simulink model "RIPS_model_pil"  (R2023a)
settings: Solver=FixedStepDiscrete  StartTime=0.0  StopTime=10  FixedStep=0.01  RelTol=1e-3
PostLoadFcn:
  | Increment = Simulink.Parameter;
  | Increment.DataType = 'uint8';
  | Increment.CoderInfo.StorageClass = 'SimulinkGlobal';
  | Increment.Value = 1;
  | 
  | SilCounterBus = Simulink.Bus;
  | SilCounterBus.Description = 'This bus contains counter inputs';
  | 
  | e1 = Simulink.BusElement;
  | e1.DataType = 'boolean';
  | e1.Name = 'ticks_to_count';
  | 
  | e2 = Simulink.BusElement;
  | e2.DataType = 'boolean';
  | e2.Name = 'reset';
  | 
  | SilCounterBus.Elements = [e1 e2];
  | clear e1 e2
  | 
  | % Step size
  | T=0.1;
  | 
  | % Input values
  | ticks_to_count.time = (0:100)'*T;
  | ticks_to_count.signals.values = boolean((floor( (0:100)/2)==(0:100)/2)');
  | ticks_to_count.signals.dimensions = 1;
  | 
  | reset.time = (0:100)'*T;
  | reset_values = boolean(zeros(101,1)); reset_values(20)=true;
  | reset.signals.values = reset_values;
  | clear reset_values
  | reset.signals.dimensions = 1;
libraries: simulink x3, rllib x1
CloseFcn:
  | clear Increment
  | clear reset
  | clear SilCounterBus
  | clear T
  | clear ticks_to_count
Description:
  | Processor-in-the-Loop Code Verification
settings Model: ModifiedByFormat=The MathWorks Inc.  SILPILSystemUnderTest=refmodels  ExtModeTrigDuration=2  Creator=The MathWorks, Inc.  LastModifiedBy=The MathWorks Inc.
settings SolverCC: PositivePriorityOrder=on  AutoInsertRateTranBlk=on
settings DataIOCC: SaveFormat=StructureWithTime  SaveOutput=off  SaveTime=off  SignalLoggingName=logsOut
settings OptimizationCC: UseDivisionForNetSlopeComputation=UseDivisionForReciprocalsOfIntegersOnly  EnhancedBackFolding=on  BooleansAsBitfields=on  PassReuseOutputArgsAs=Individual arguments  ExpressionDepthLimit=2147483647  StateBitsets=on  DataBitsets=on  ZeroExternalMemoryAtStartup=off  ZeroInternalMemoryAtStartup=off  NoFixptDivByZeroProtection=on  EfficientFloat2IntCast=on  LifeSpan=1  MaxStackSize=64  SimCompilerOptimization=on  EfficientTunableParamExpr=on
settings DebuggingCC: ReadBeforeWriteMsg=DisableAll  WriteAfterWriteMsg=DisableAll  WriteAfterReadMsg=DisableAll  UnderspecifiedInitializationDetection=Classic  CheckExecutionContextPreStartOutputMsg=on  FcnCallInpInsideContextMsg=warning  UnconnectedInputMsg=warning  UnconnectedOutputMsg=warning  UnconnectedLineMsg=warning  UniqueDataStoreMsg=error  AllowSymbolicDim=off  ModelReferenceSymbolNameMessage=none  StateNameClashWarn=warning  StrictBusMsg=ErrorOnBusTreatedAsVector  SFUnexpectedBacktrackingDiag=warning  SFNoUnconditionalDefaultTransitionDiag=warning  SFExecutionAtInitializationDiag=none  ArithmeticOperatorsInVariantConditions=warning
settings HardwareCC: ProdBitPerInt=16  ProdBitPerPointer=16  ProdBitPerSizeT=16  ProdBitPerPtrDiffT=16  ProdLargestAtomicFloat=None  ProdWordSize=8  ProdHWDeviceType=Atmel->AVR  TargetHWDeviceType=Generic->32-bit Embedded Processor
settings ModelReferenceCC: EnableRefExpFcnMdlSchedulingChecks=on  CheckModelReferenceTargetMessage=none  PropagateSignalLabelsOutOfModel=off
settings SFSimCC: SimUseLocalCustomCode=off  MATLABDynamicMemAlloc=off  CustomCodeUndefinedFunction=UseInterfaceOnly
settings RTWCC: Description=Embedded Coder  SystemTargetFile=ert.tlc  HardwareBoard=Arduino Mega 2560  TemplateMakefile=ert_default_tmf  GenerateReport=on  RTWVerbose=off  RTWUseLocalCustomCode=off  Toolchain=Arduino AVR  BuildConfiguration=Faster Runs  IncludeHyperlinkInReport=on  PortableWordSizes=on  CodeProfilingSaveOptions=AllData  GenerateTraceInfo=on  GenerateTraceReport=on  GenerateTraceReportSl=on  GenerateTraceReportSf=on  GenerateTraceReportEml=on  GenerateCodeMetricsReport=on
settings CodeAppCC: ForceParamTrailComments=on  IgnoreCustomStorageClasses=off  SimulinkDataObjDesc=on  CustomSymbolStrGlobalVar=rt$N$M  CustomSymbolStrType=$N$M  CustomSymbolStrFcn=$N$M$F  CustomSymbolStrModelFcn=$N  CustomSymbolStrMacro=$N$M  InsertBlockDesc=on  StateflowObjectComments=on  InternalIdentifier=Classic
settings ERTTargetCC: UtilityFuncGeneration=Shared location  MultiwordLength=2048  IncludeMdlTerminateFcn=off  CombineSignalStateStructs=on  SupportNonFinite=off  SupportComplex=off  SupportContinuousTime=on  SupportVariableSizeSignals=on  ERTFilePackagingFormat=CompactWithDataFile  ConvertIfToSwitch=off  SuppressUnreachableDefaultCases=off
settings ConfigComp: CovMetricSettings=dw  CovSaveCumulativeToWorkspaceVar=on  CovSaveSingleToWorkspaceVar=on  CovExternalEMLEnable=off  CovSFcnEnable=off

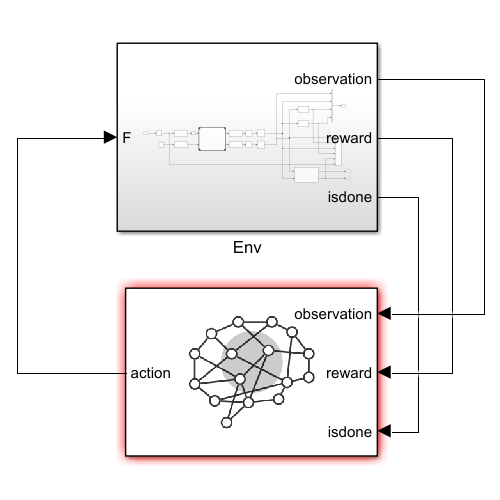
[thumbnail: Simulink's stored preview of the top-level diagram]
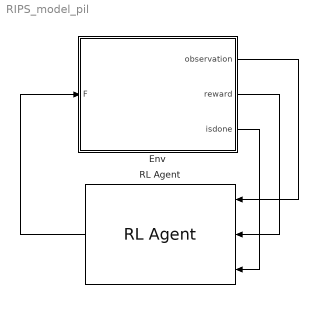
== system RIPS_model_pil ==
  Env : Subsystem
  RL Agent : rllib/RL Agent  Agent=agent  ExternalActionAsInput=off  ProvideLastAction=off  ProvideCumRwd=off  TreatAsDirectFeedthrough=on  UseStrictObservationDataTypes=off
  wires:
  Env/1(observation) -> RL Agent/1
  Env/2(reward) -> RL Agent/2
  Env/3(isdone) -> RL Agent/3
  RL Agent/1 -> Env/1(F)

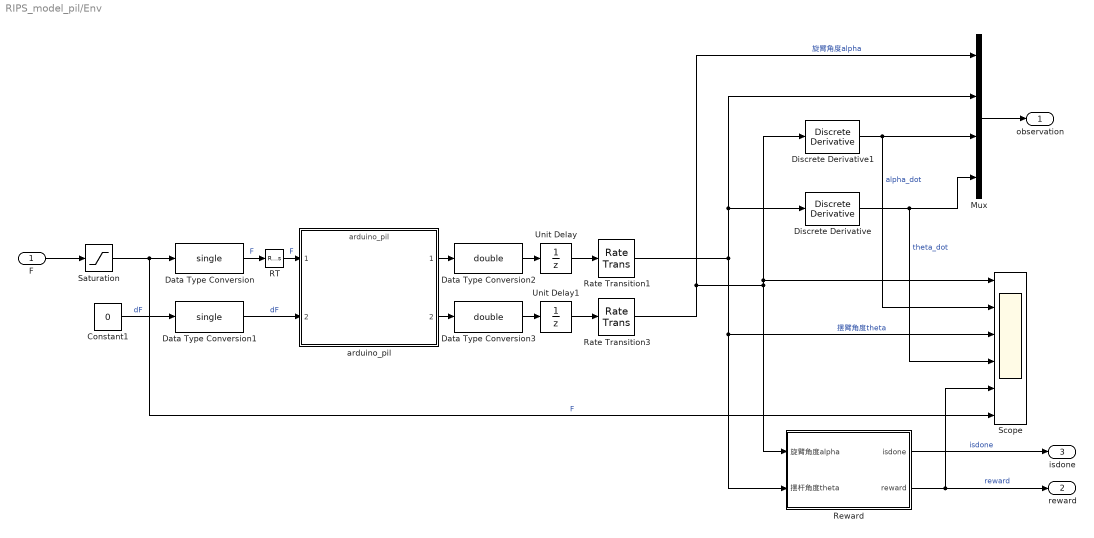
== system RIPS_model_pil/Env ==
  F : Inport
  Constant1 : Constant  Value=0
  Data Type Conversion : DataTypeConversion  OutDataTypeStr=single  SaturateOnIntegerOverflow=off  RndMeth=Floor
  Data Type Conversion1 : DataTypeConversion  OutDataTypeStr=single  SaturateOnIntegerOverflow=off  RndMeth=Floor
  Data Type Conversion2 : DataTypeConversion  OutDataTypeStr=double  SaturateOnIntegerOverflow=off  RndMeth=Floor
  Data Type Conversion3 : DataTypeConversion  OutDataTypeStr=double  SaturateOnIntegerOverflow=off  RndMeth=Floor
  Discrete Derivative : simulink/Discrete/Discrete Derivative  gainval=1.0  ICPrevScaledInput=0  OutMin=[]  OutMax=[]  OutDataType=fixdt(1, 16)  OutScaling=2^-10  DoSatur=off
  Discrete Derivative1 : simulink/Discrete/Discrete Derivative  gainval=1.0  ICPrevScaledInput=0  OutMin=[]  OutMax=[]  OutDataType=fixdt(1, 16)  OutScaling=2^-10  DoSatur=off
  Mux : Mux
  RT : RateTransition  Integrity=off  OutPortSampleTimeOpt=Inherit  OutPortSampleTime=0.02
  Rate Transition1 : RateTransition  Integrity=off  OutPortSampleTimeOpt=Inherit
  Rate Transition3 : RateTransition
  Reward : Subsystem
  Saturation : Saturate  UpperLimit=10  LowerLimit=-10
  Scope : Scope  NumInputPorts=6
  Unit Delay : UnitDelay  SampleTime=-1  HasFrameUpgradeWarning=on
  Unit Delay1 : UnitDelay  SampleTime=-1  HasFrameUpgradeWarning=on
  arduino_pil : ModelReference  ModelNameDialog=arduino_pil.slx  SimulationMode=Processor-in-the-loop (PIL)  ModelReferenceVersion=8.51
  observation : Outport
  reward : Outport  Port=2
  isdone : Outport  Port=3
  wires:
  Constant1/1 -> Data Type Conversion1/1  "dF"
  Discrete Derivative/1 -> Mux/4, Scope/4  "theta_dot"
  Reward/2(reward) -> reward/1, Scope/5  "reward"
  Discrete Derivative1/1 -> Mux/3, Scope/2  "alpha_dot"
  Data Type Conversion3/1 -> Unit Delay1/1
  Mux/1 -> observation/1
  F/1 -> Saturation/1
  Saturation/1 -> Scope/6, Data Type Conversion/1  "F"
  Reward/1(isdone) -> isdone/1  "isdone"
  Data Type Conversion/1 -> RT/1  "F"
  Data Type Conversion1/1 -> arduino_pil/2  "dF"
  RT/1 -> arduino_pil/1  "F"
  arduino_pil/1 -> Data Type Conversion2/1
  arduino_pil/2 -> Data Type Conversion3/1
  Rate Transition1/1 -> Mux/2, Discrete Derivative/1, Reward/2(摆杆角度theta), Scope/3  "摆臂角度theta"
  Rate Transition3/1 -> Mux/1, Scope/1, Discrete Derivative1/1, Reward/1(旋臂角度alpha)  "旋臂角度alpha"
  Data Type Conversion2/1 -> Unit Delay/1
  Unit Delay/1 -> Rate Transition1/1
  Unit Delay1/1 -> Rate Transition3/1

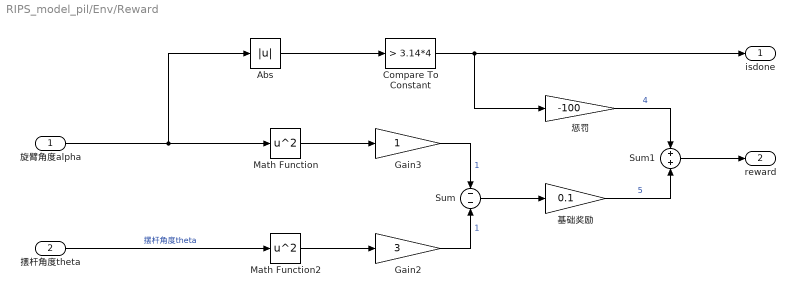
== system RIPS_model_pil/Env/Reward ==
  旋臂角度alpha : Inport
  摆杆角度theta : Inport  Port=2
  Abs : Abs  SaturateOnIntegerOverflow=off
  Compare To Constant : simulink/Logic and Bit Operations/Compare To Constant  relop=>  const=3.14*4  OutDataTypeStr=boolean
  Gain2 : Gain  Gain=3
  Gain3 : Gain
  Math Function : Math  Operator=square  SignedPower=on
  Math Function2 : Math  Operator=square  SignedPower=on
  Sum : Sum  Inputs=--
  Sum1 : Sum
  基础奖励 : Gain  Gain=0.1
  惩罚 : Gain  Gain=-100
  isdone : Outport
  reward : Outport  Port=2
  wires:
  基础奖励/1 -> Sum1/2  "5"
  Sum/1 -> 基础奖励/1
  惩罚/1 -> Sum1/1  "4"
  Gain3/1 -> Sum/1  "1"
  Abs/1 -> Compare To Constant/1
  Math Function/1 -> Gain3/1
  Sum1/1 -> reward/1
  旋臂角度alpha/1 -> Abs/1, Math Function/1
  Compare To Constant/1 -> isdone/1, 惩罚/1
  摆杆角度theta/1 -> Math Function2/1  "摆杆角度theta"
  Math Function2/1 -> Gain2/1
  Gain2/1 -> Sum/2  "1"
